simulink model "flightController"  (R2026a)
settings: Solver=ode3  StartTime=0  FixedStep=Ts  EnableMultiTasking=on
settings Model: Creator=The MathWorks, Inc.  LastModifiedBy=The MathWorks, Inc.
settings OptimizationCC: BufferReuse=off
settings DebuggingCC: SymbolicDimsDataTypeCodeGenerationDiagnostic=none
settings HardwareCC: ProdHWDeviceType=32-bit Generic

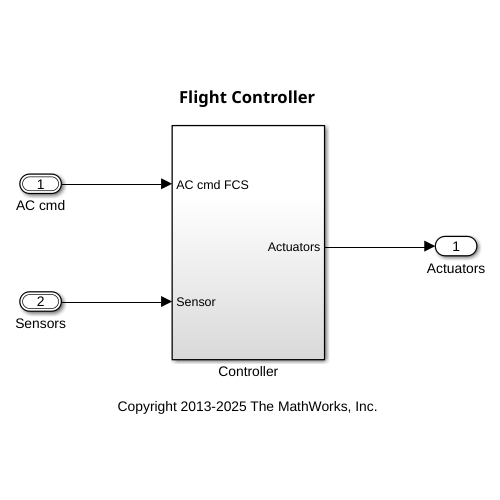
[thumbnail: Simulink's stored preview of the top-level diagram]
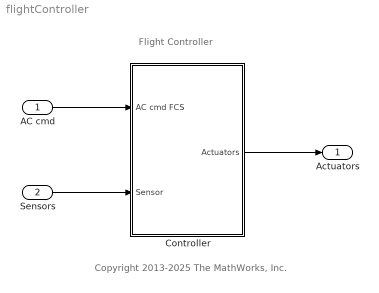
== system flightController ==
  note: Copyright 2013-2025 The MathWorks, Inc.
  note: Flight Controller
  AC cmd : Inport  OutDataTypeStr=Bus: CommandBus
  Sensors : Inport  Port=2  OutDataTypeStr=Bus: SensorsBus  BusOutputAsStruct=on
  Controller : Subsystem
  Actuators : Outport  VectorParamsAs1DForOutWhenUnconnected=off
  wires:
  AC cmd/1 -> Controller/1(AC cmd FCS)
  Sensors/1 -> Controller/2(Sensor)
  Controller/1(Actuators) -> Actuators/1

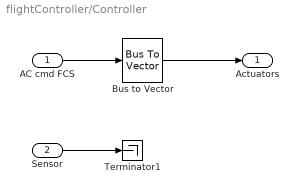
== system flightController/Controller ==
  AC cmd FCS : Inport
  Sensor : Inport  Port=2
  Bus to Vector : BusToVector
  Terminator1 : Terminator
  Actuators : Outport  VectorParamsAs1DForOutWhenUnconnected=off
  wires:
  Sensor/1 -> Terminator1/1
  Bus to Vector/1 -> Actuators/1
  AC cmd FCS/1 -> Bus to Vector/1
